simulink model "DCHR_A46_Compressor_Closed_Loop"  (R2026a)
settings: Solver=FixedStepDiscrete  StopTime=603900  FixedStep=900
settings Model: Creator=Lysda  LastModifiedBy=Lysda

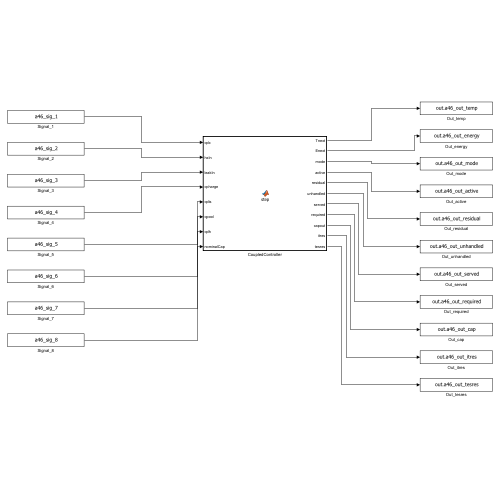
[thumbnail: Simulink's stored preview of the top-level diagram]
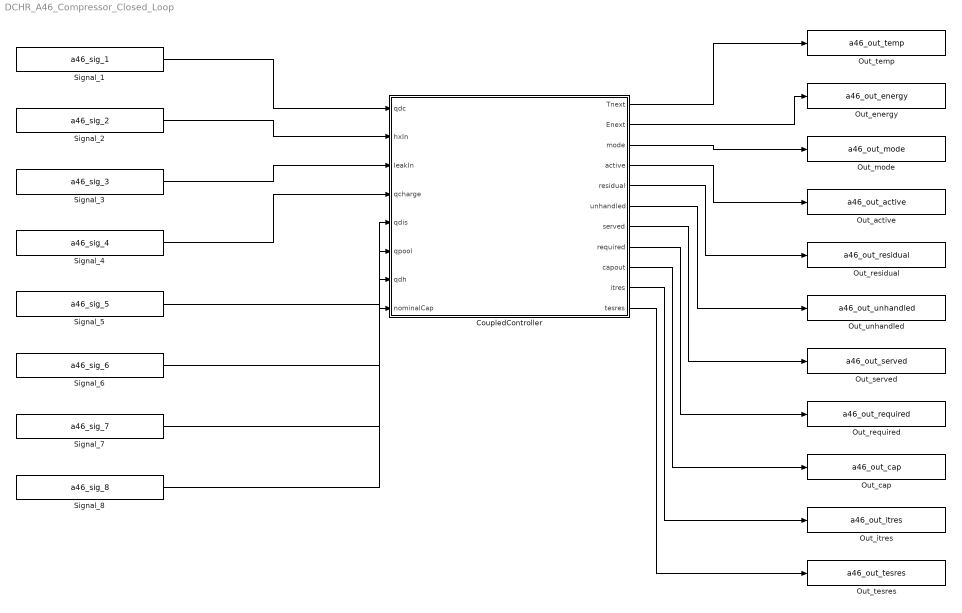
== system DCHR_A46_Compressor_Closed_Loop ==
  CoupledController : MATLAB Function  TreatAsAtomicUnit=on
  Out_active : ToWorkspace  VariableName=a46_out_active  SampleTime=-1
  Out_cap : ToWorkspace  VariableName=a46_out_cap  SampleTime=-1
  Out_energy : ToWorkspace  VariableName=a46_out_energy  SampleTime=-1
  Out_itres : ToWorkspace  VariableName=a46_out_itres  SampleTime=-1
  Out_mode : ToWorkspace  VariableName=a46_out_mode  SampleTime=-1
  Out_required : ToWorkspace  VariableName=a46_out_required  SampleTime=-1
  Out_residual : ToWorkspace  VariableName=a46_out_residual  SampleTime=-1
  Out_served : ToWorkspace  VariableName=a46_out_served  SampleTime=-1
  Out_temp : ToWorkspace  VariableName=a46_out_temp  SampleTime=-1
  Out_tesres : ToWorkspace  VariableName=a46_out_tesres  SampleTime=-1
  Out_unhandled : ToWorkspace  VariableName=a46_out_unhandled  SampleTime=-1
  Signal_1 : FromWorkspace  VariableName=a46_sig_1
  Signal_2 : FromWorkspace  VariableName=a46_sig_2
  Signal_3 : FromWorkspace  VariableName=a46_sig_3
  Signal_4 : FromWorkspace  VariableName=a46_sig_4
  Signal_5 : FromWorkspace  VariableName=a46_sig_5
  Signal_6 : FromWorkspace  VariableName=a46_sig_6
  Signal_7 : FromWorkspace  VariableName=a46_sig_7
  Signal_8 : FromWorkspace  VariableName=a46_sig_8
  wires:
  Signal_1/1 -> CoupledController/1(qdc)
  Signal_2/1 -> CoupledController/2(hxIn)
  Signal_3/1 -> CoupledController/3(leakIn)
  Signal_4/1 -> CoupledController/4(qcharge)
  Signal_5/1 -> CoupledController/5(qdis)
  Signal_6/1 -> CoupledController/6(qpool)
  Signal_7/1 -> CoupledController/7(qdh)
  Signal_8/1 -> CoupledController/8(nominalCap)
  CoupledController/1(Tnext) -> Out_temp/1
  CoupledController/2(Enext) -> Out_energy/1
  CoupledController/3(mode) -> Out_mode/1
  CoupledController/4(active) -> Out_active/1
  CoupledController/5(residual) -> Out_residual/1
  CoupledController/6(unhandled) -> Out_unhandled/1
  CoupledController/7(served) -> Out_served/1
  CoupledController/8(required) -> Out_required/1
  CoupledController/9(capout) -> Out_cap/1
  CoupledController/10(itres) -> Out_itres/1
  CoupledController/11(tesres) -> Out_tesres/1

== matlab function DCHR_A46_Compressor_Closed_Loop/CoupledController ==
  data: qdc input; Tnext output; hxIn input; leakIn input; qcharge input; qdis input; qpool input; qdh input; nominalCap input; Enext output; mode output; active output; residual output; unhandled output; served output; required output; capout output; itres output; tesres output
function [Tnext,Enext,mode,active,residual,unhandled,served,required,capout,itres,tesres] = step(qdc,hxIn,leakIn,qcharge,qdis,qpool,qdh,nominalCap)
%#codegen
persistent E T state prevActive prevShed pending good res lastTrip effCap hpAvailable
if isempty(E)
 E=450*3.6e6;T=30;state=0;prevActive=0;prevShed=0;pending=0;good=0;res=0;lastTrip=false;effCap=330000;hpAvailable=0;
end
dt=900;Emax=900*3.6e6;
effCap=min(nominalCap,effCap+60000);
fault=nominalCap<=0 || T>=42;
if (state==0 || state==3) && fault
 state=1;pending=0;
end
if state==1 && ~fault && T<36
 state=0;pending=0;
end
if state==1
 if pending<2
  active=qdc;pending=pending+1;
 else
  state=2;active=0;good=0;
 end
elseif state==2
 active=0;
 if nominalCap>0 && T<36
  good=good+1;
 else
  good=0;
 end
 if good>=2
  state=3;active=min(qdc,15000);
 end
elseif state==3
 active=min(qdc,prevActive+15000);
 if active>=qdc-1e-8
  state=0;
 end
else
 h0=min(hxIn,qdc);l0=min(leakIn,max(0,qdc-h0));
 av0=max(0,qdc-h0-l0);
 demand=qpool+qdh;loss0=.002*E/86400;
 dcap0=max(0,(E-dt*loss0)*.91/dt);
 dis0=min([qdis,demand,dcap0]);
 room0=max(0,(Emax-E+dt*(dis0/.91+loss0))/(dt*.93));
 charge0=min(qcharge,room0);
 need0=max(0,demand-dis0);desired0=need0+charge0;
 cop0=max(2,min(5,3.5+.04*(T-30)));
 source0=min(av0,desired0*(cop0-1)/cop0);
 required0=max(0,qdc-h0-l0-source0);
 target=min(.4*qdc,max(0,required0-effCap));
 shed=min(target,prevShed+15000);
 active=qdc-shed;
end
if state==2 && ~lastTrip
 res=.12*prevActive;
elseif res>0
 res=res*exp(-dt/3600);
end
active=min(active,max(0,qdc-res));
qit=active+res;
hx=min(hxIn,qit);leak=min(leakIn,max(0,qit-hx));
available=max(0,qit-hx-leak);
demand=qpool+qdh;loss=.002*E/86400;
discap=max(0,(E-dt*loss)*.91/dt);
dis=min([qdis,demand,discap]);
room=max(0,(Emax-E+dt*(dis/.91+loss))/(dt*.93));
creq=min(qcharge,room);need=max(0,demand-dis);
desired=need+creq;cop=max(2,min(5,3.5+.04*(T-30)));
sourceTarget=min(available,desired*(cop-1)/cop);
hpAvailable=hpAvailable+(1-exp(-dt/1800))*(sourceTarget-hpAvailable);
source=min(sourceTarget,hpAvailable);
power=source/(cop-1);cond=source+power;
servedhp=min(need,cond);charge=min(creq,max(0,cond-servedhp));
served=dis+servedhp;
Enext=max(0,min(Emax,E+dt*(.93*charge-dis/.91-loss)));
required=max(0,qit-hx-leak-source);
rejected=min(required,effCap);
unhandled=max(0,required-rejected);
passive=2000*max(0,T-30);
Tnext=max(30,T+dt*(unhandled-passive)/8e6);
itres=qit-hx-leak-source-rejected-unhandled;
tesres=Enext-E-dt*(.93*charge-dis/.91-loss);
mode=state;residual=res;capout=effCap;
E=Enext;T=Tnext;prevActive=active;prevShed=qdc-active;lastTrip=(state==2);
end
